simulink model "CSTR_ClosedLoop"  (R2026b)
settings: Solver=ode45  StartTime=0  StopTime=5  EnableMultiTasking=on
libraries: mpclib x1
settings Model: FPTRunName=Active  Creator=The MathWorks, Inc.  LastModifiedBy=thomschu
settings DataIOCC: ExternalInput=getinputstruct(op_trim1)  InitialState=getstatestruct(op_trim1)  LimitDataPoints=on  LoadExternalInput=on  LoadInitialState=on  ReturnWorkspaceOutputs=off  SaveFormat=Array  SignalLoggingName=logsOut
settings OptimizationCC: BooleanDataType=off  BufferReuse=off  DefaultParameterBehavior=Inlined  EfficientMapNaN2IntZero=off  InlineInvariantSignals=on  LifeSpan=inf  MemsetInitFltsAndDblsToZero=off
settings DebuggingCC: AlgebraicLoopMsg=none  ArithmeticOperatorsInVariantConditions=warning  CheckExecutionContextPreStartOutputMsg=on  FcnCallInpInsideContextMsg=warning  MergeDetectMultiDrivingBlocksExec=none  MultiTaskCondExecSysMsg=none  MultiTaskDSMMsg=warning  SFExecutionAtInitializationDiag=none  SFNoUnconditionalDefaultTransitionDiag=warning  SFUnexpectedBacktrackingDiag=warning  SaveWithParameterizedLinksMsg=none  SignalResolutionControl=TryResolveAllWithWarning  StateNameClashWarn=warning
settings HardwareCC: ProdEndianess=Unspecified  ProdHWDeviceType=32-bit Generic  ProdIntDivRoundTo=Undefined  ProdLargestAtomicFloat=None  TargetUnknown=on
settings ModelReferenceCC: PropagateSignalLabelsOutOfModel=off
settings SFSimCC: CustomCodeUndefinedFunction=UseInterfaceOnly  SimUseLocalCustomCode=off
settings RTWCC: DLArmComputeVersion=19.05  RTWUseLocalCustomCode=off
settings CodeAppCC: StateflowObjectComments=on
settings GRTTargetCC: CombineOutputUpdateFcns=off  GRTInterface=on  TargetFcnLib=ansi_tfl_tmw.mat  TargetLangStandard=C89/C90 (ANSI)
settings ConfigComp: CovExternalEMLEnable=off  CovSaveCumulativeToWorkspaceVar=on  CovSaveSingleToWorkspaceVar=on

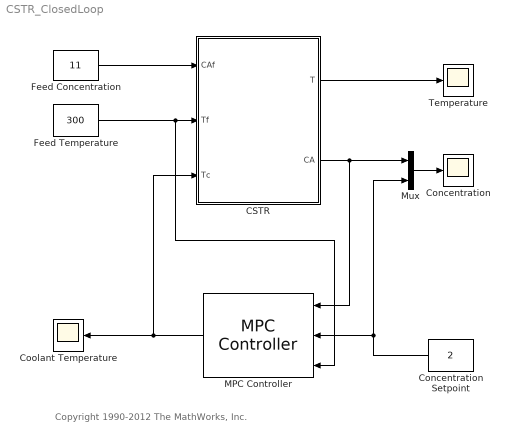
== system CSTR_ClosedLoop ==
  note: Copyright 1990-2012 The MathWorks, Inc.
  CSTR : Subsystem
  Concentration : Scope
      settings: ActiveDisplayYMinimum=1.5481179472007078  ActiveDisplayYMaximum=2.1704160894301743
  Concentration Setpoint : Constant  Value=2  SampleTime=0
  Coolant Temperature : Scope
      settings: ActiveDisplayYMinimum=280  ActiveDisplayYMaximum=320
  Feed Concentration : Constant  Value=11  SampleTime=0
  Feed Temperature : Constant  Value=300  SampleTime=0
  MPC Controller : mpclib/MPC Controller  mpcobj=mpc1  x0=[]  is_multiple=0  enable_value=0  return_u0=off  updateMPCinCallerWorkspace=on  md_inport=on  mv_inport=off  uref_inport=off  return_cost=off  return_mvseq=off  return_qpstatus=off  return_xseq=off  return_state=off  return_ovseq=off  state_inport=off  umin_inport=off  umax_inport=off  ymin_inport=off  ymax_inport=off  cc_inport=off  ywt_inport=off  uwt_inport=off  duwt_inport=off  rhoeps_inport=off  pm_inport=off  MaximumP=10  HorizonChoice=FixedHorizon  n_ts=0.1  n_p=20  n_mv=1  n_md=1  n_ud=1  n_mo=1  n_uo=0  BlockDataType=double  SampleTimeInherited=off  switch_inport=off
  Mux : Mux  Inputs=2
  Temperature : Scope
      settings: ActiveDisplayYMinimum=280  ActiveDisplayYMaximum=320  DataLoggingVariableName=ScopeData2
  wires:
  Feed Concentration/1 -> CSTR/1(CAf)
  CSTR/2(CA) -> Mux/1, MPC Controller/1
  Mux/1 -> Concentration/1
  MPC Controller/1 -> CSTR/3(Tc), Coolant Temperature/1
  Concentration Setpoint/1 -> MPC Controller/2, Mux/2
  Feed Temperature/1 -> MPC Controller/3, CSTR/2(Tf)
  CSTR/1(T) -> Temperature/1

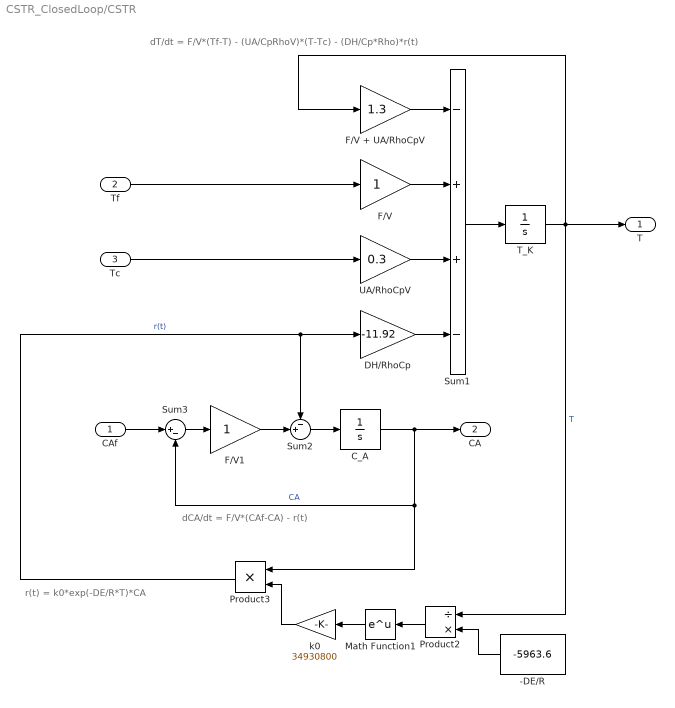
== system CSTR_ClosedLoop/CSTR ==
  note: dT/dt = F/V*(Tf-T) - (UA/CpRhoV)*(T-Tc) - (DH/Cp*Rho)*r(t)
  note: r(t) = k0*exp(-DE/R*T)*CA
  note: dCA/dt = F/V*(CAf-CA) - r(t)
  CAf : Inport
  Tf : Inport  Port=2
  Tc : Inport  Port=3
  -DE/R : Constant  Value=-5963.6  SampleTime=0
  C_A : Integrator  InitialCondition=8.5695  LimitOutput=on  LowerSaturationLimit=0
  DH/RhoCp : Gain  Gain=-11.92  SaturateOnIntegerOverflow=on  OutDataTypeStr=Inherit: Same as input  ParamDataTypeStr=Inherit: Same as input
  F/V : Gain  SaturateOnIntegerOverflow=on  OutDataTypeStr=Inherit: Same as input  ParamDataTypeStr=Inherit: Same as input
  F/V + UA/RhoCpV : Gain  Gain=1.3  SaturateOnIntegerOverflow=on  OutDataTypeStr=Inherit: Same as input  ParamDataTypeStr=Inherit: Same as input
  F/V1 : Gain  SaturateOnIntegerOverflow=on  OutDataTypeStr=Inherit: Same as input  ParamDataTypeStr=Inherit: Same as input
  Math Function1 : Math  SignedPower=on
  Product2 : Product  Inputs=/*  InputSameDT=on  RndMeth=Zero  SaturateOnIntegerOverflow=on  OutDataTypeStr=Inherit: Same as first input
  Product3 : Product  InputSameDT=on  RndMeth=Zero  SaturateOnIntegerOverflow=on  OutDataTypeStr=Inherit: Same as first input
  Sum1 : Sum  Inputs=-++-  InputSameDT=on  SaturateOnIntegerOverflow=on  OutDataTypeStr=Inherit: Same as first input
  Sum2 : Sum  Inputs=-+|
  Sum3 : Sum  Inputs=|+-
  T_K : Integrator  InitialCondition=311.267  LimitOutput=on  LowerSaturationLimit=0
  UA/RhoCpV : Gain  Gain=0.3  SaturateOnIntegerOverflow=on  OutDataTypeStr=Inherit: Same as input  ParamDataTypeStr=Inherit: Same as input
  k0 : Gain  Gain=34930800  SaturateOnIntegerOverflow=on  OutDataTypeStr=Inherit: Same as input  ParamDataTypeStr=Inherit: Same as input
  T : Outport
  CA : Outport  Port=2
  wires:
  UA/RhoCpV/1 -> Sum1/3
  F/V/1 -> Sum1/2
  F/V + UA/RhoCpV/1 -> Sum1/1
  k0/1 -> Product3/2
  Product2/1 -> Math Function1/1
  Math Function1/1 -> k0/1
  -DE/R/1 -> Product2/2
  T_K/1 -> T/1, F/V + UA/RhoCpV/1, Product2/1  "T"
  Sum2/1 -> C_A/1
  F/V1/1 -> Sum2/2
  Sum3/1 -> F/V1/1
  CAf/1 -> Sum3/1
  DH/RhoCp/1 -> Sum1/4
  Sum1/1 -> T_K/1
  Product3/1 -> DH/RhoCp/1, Sum2/1  "r(t)"
  C_A/1 -> Sum3/2, Product3/1, CA/1  "CA"
  Tf/1 -> F/V/1
  Tc/1 -> UA/RhoCpV/1
